simulink model "AGC_script"  (R2024b)
settings: Solver=VariableStepAuto  StartTime=0.0  StopTime=simTim  RelTol=1e-3
libraries: audiomeasurements x3, commrfcorlib x1, dspvision x1
settings Model: Creator=Pedro  LastModifiedBy=Pedro

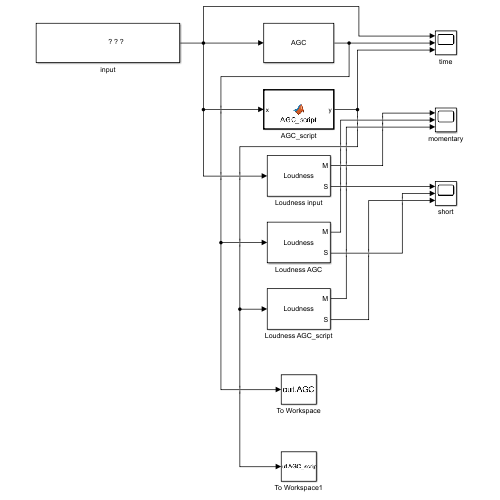
[thumbnail: Simulink's stored preview of the top-level diagram]
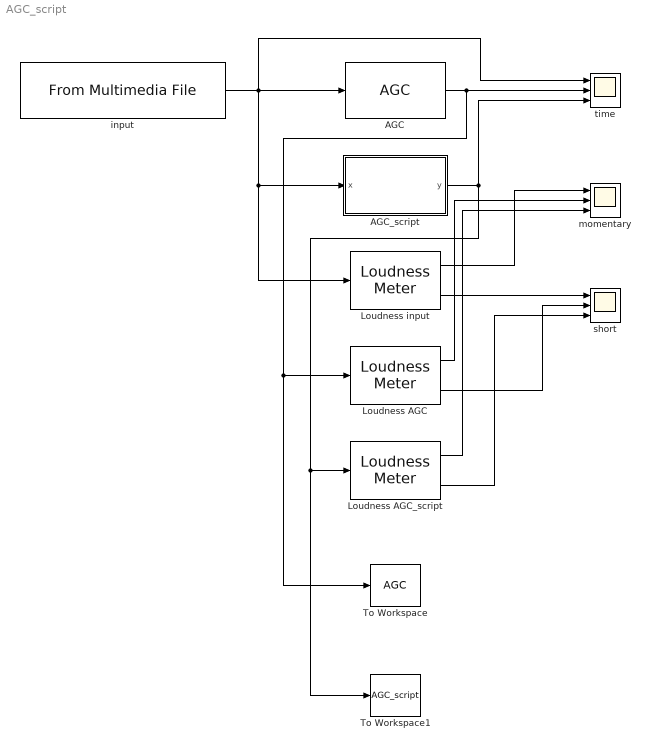
== system AGC_script ==
  AGC : commrfcorlib/AGC  LegacyMode=off  DetectorMethod=Rectifier  LoopMethod=Linear  UpdatePeriod=100  StepSize=0.1  AdaptationStepSize=0.1  DesiredOutputPower=0.01  AveragingLength=0.4*48000  MaximumGain=30  MaxPowerGain=15  GainOutputPort=off  InputPowerOutputPort=off  SimulateUsing=Interpreted execution
  AGC_script : MATLAB Function  TreatAsAtomicUnit=on
  Loudness AGC : audiomeasurements/Loudness Meter  ChannelWeights=[ 1, 1, 1, 1.41, 1.41 ]  UseRelativeScale=off  TargetLoudness=-23.0  OutputTruePeak=off  InheritSampleRate=off  SampleRate=48000  SimulateUsing=Interpreted execution
  Loudness AGC_script : audiomeasurements/Loudness Meter  ChannelWeights=[ 1, 1, 1, 1.41, 1.41 ]  UseRelativeScale=off  TargetLoudness=-23.0  OutputTruePeak=off  InheritSampleRate=off  SampleRate=48000  SimulateUsing=Interpreted execution
  Loudness input : audiomeasurements/Loudness Meter  ChannelWeights=[ 1, 1, 1, 1.41, 1.41 ]  UseRelativeScale=off  TargetLoudness=-23.0  OutputTruePeak=off  InheritSampleRate=off  SampleRate=48000  SimulateUsing=Interpreted execution
  To Workspace : ToWorkspace  VariableName=AGC  SampleTime=-1
      settings: Save2DSignal=2-D array (concatenate along first dimension)
  To Workspace1 : ToWorkspace  VariableName=AGC_script  SampleTime=-1
      settings: Save2DSignal=2-D array (concatenate along first dimension)
  input : dspvision/From Multimedia File  inputFilename=input_track_path  readRange=[1 Inf]  loop=on  numPlays=inf  outputStreams=Audio only  videoDataType=single  audioDataType=double  inheritSampleTime=on  userDefinedSampleTime=1/30  noAudioOutput=off  isIntensityVideo=off  fourcc=RGB  colorVideoFormat=Separate color signals  outputEOF=off  dataOrg=Column-major  audioFrameSize=1024  computeAudioFrameSize=off  outSamplingMode=Sample based
      settings: LibrarySourceBlock=audiosources/From Multimedia File
  momentary : Scope  NumInputPorts=3
  short : Scope  NumInputPorts=3
  time : Scope  NumInputPorts=3
  wires:
  input/1 -> time/1, AGC/1, AGC_script/1(x), Loudness input/1
  AGC_script/1(y) -> time/3, To Workspace1/1, Loudness AGC_script/1
  AGC/1 -> To Workspace/1, Loudness AGC/1, time/2
  Loudness input/1 -> momentary/1
  Loudness AGC/1 -> momentary/2
  Loudness AGC_script/1 -> momentary/3
  Loudness input/2 -> short/1
  Loudness AGC/2 -> short/2
  Loudness AGC_script/2 -> short/3

== matlab function AGC_script/AGC_script ==
  data: x input; y output
function y  = AGC_script(x)

persistent gain buffer bufferSum bufferIdx;

ref = -20;                  % Reference (dB)
fs = 48000;                 % Sampling frequency (Hz)
winLength = round(0.4*fs);  % Averaging window length (400ms)
stepSize = 0.1;             % step size
maxGain = 10;               % Maximum gain (dB)
silence = -50;              % What's considered silende (dB)

if isempty(gain)
    gain = 0;                     % dB gain
    buffer = ones(winLength, 1);  % Circular buffer
    bufferSum = winLength;        % Running sum of buffer
    bufferIdx = 1;                % Buffer index
end

y = zeros(length(x),1);

for n = 1:length(x)

    % moving average
    if abs(x(n)) > 10^(silence/20)
        bufferSum = bufferSum - buffer(bufferIdx) + x(n)^2;
        buffer(bufferIdx) = x(n)^2;
        bufferIdx = mod(bufferIdx,winLength) + 1;
    end

    y(n) = x(n) * exp(gain);
    y(n) = max(min(y(n),1),-1);
  
    pow = bufferSum/winLength;
    pow = max(pow,eps);

    e = log(10^(ref/10)) - (log(pow) + 2*gain);

    gain = gain + stepSize * e;
    gain = min(gain,maxGain);
end

end
